simulink model "SistemaP4"  (R2020b)
settings: Solver=ode15s  StartTime=0  StopTime=10  MaxStep=1E-2  RelTol=1e-3
libraries: fl_lib x14, nesl_utility x6, pid_lib x1
settings Model: Creator=ggjai  LastModifiedBy=ggjai
settings SolverCC: AlgebraicLoopSolver=LineSearch
settings DataIOCC: SaveFormat=Array  SaveOutput=off  SignalLogging=off  DSMLogging=off  ReturnWorkspaceOutputs=off  TimeSaveName=t
settings DebuggingCC: AlgebraicLoopMsg=none  ArtificialAlgebraicLoopMsg=none  MaxConsecutiveZCsMsg=none  ModelReferenceExtraNoncontSigs=none  OperatingPointInterfaceChecksumMismatchMsg=none

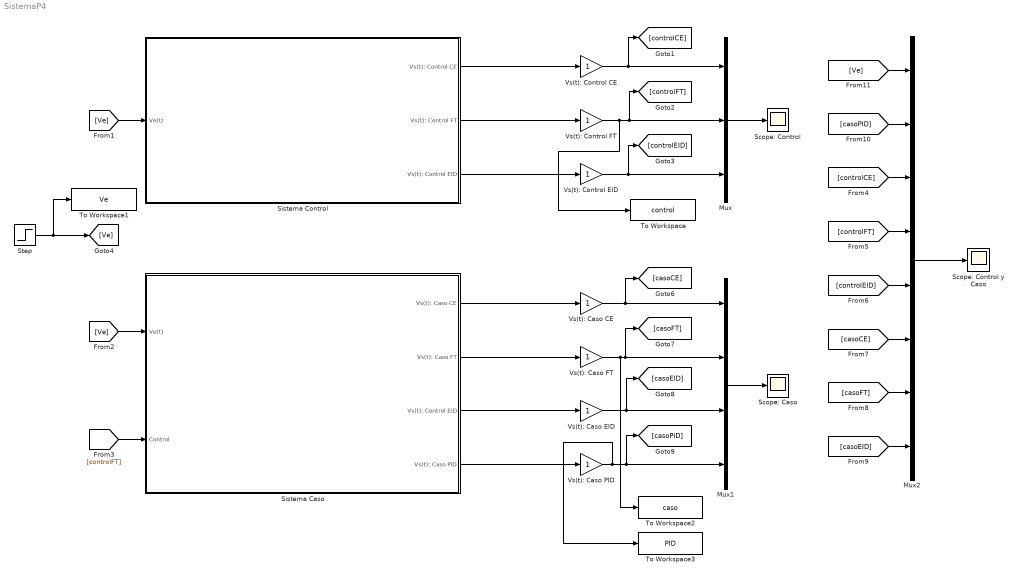
== system SistemaP4 ==
  Mux : Mux  Inputs=3
  Mux1 : Mux
  Mux2 : Mux  Inputs=8
  Scope: Caso : Scope
  Scope: Control : Scope
  Scope: Control y Caso : Scope
  Sistema Caso : Subsystem
  Sistema Control : Subsystem
  Step : Step  SampleTime=0
  To Workspace : ToWorkspace  VariableName=control  SampleTime=-1
  To Workspace1 : ToWorkspace  VariableName=Ve  SampleTime=-1
  To Workspace2 : ToWorkspace  VariableName=caso  SampleTime=-1
  To Workspace3 : ToWorkspace  VariableName=PID  SampleTime=-1
  Vs(t): Caso CE : Gain
  Vs(t): Caso EID : Gain
  Vs(t): Caso FT : Gain
  Vs(t): Caso PID : Gain
  Vs(t): Control CE : Gain
  Vs(t): Control EID : Gain
  Vs(t): Control FT : Gain
  wires:
  [Ve] -> Sistema Control/1(Ve(t))
  Mux/1 -> Scope: Control/1
  Step/1 -> To Workspace1/1, [Ve]
  Sistema Control/3(Vs(t): Control EID) -> Vs(t): Control EID/1
  Vs(t): Control EID/1 -> [controlEID], Mux/3
  Vs(t): Control FT/1 -> To Workspace/1, [controlFT], Mux/2
  Sistema Control/2(Vs(t): Control FT) -> Vs(t): Control FT/1
  Sistema Control/1(Vs(t): Control CE) -> Vs(t): Control CE/1
  Vs(t): Control CE/1 -> [controlCE], Mux/1
  [Ve] -> Sistema Caso/1(Ve(t))
  Mux1/1 -> Scope: Caso/1
  Vs(t): Caso CE/1 -> [casoCE], Mux1/1
  Vs(t): Caso FT/1 -> To Workspace2/1, [casoFT], Mux1/2
  Vs(t): Caso EID/1 -> [casoEID], Mux1/3
  Sistema Caso/1(Vs(t): Caso CE) -> Vs(t): Caso CE/1
  Sistema Caso/2(Vs(t): Caso FT) -> Vs(t): Caso FT/1
  Sistema Caso/3(Vs(t): Control EID) -> Vs(t): Caso EID/1
  Mux2/1 -> Scope: Control y Caso/1
  Sistema Caso/4(Vs(t): Caso PID) -> Vs(t): Caso PID/1
  Vs(t): Caso PID/1 -> To Workspace3/1, Mux1/4, [casoPID]
  [controlFT] -> Sistema Caso/2(Control)
  [casoEID] -> Mux2/8
  [casoFT] -> Mux2/7
  [casoCE] -> Mux2/6
  [controlEID] -> Mux2/5
  [controlFT] -> Mux2/4
  [controlCE] -> Mux2/3
  [casoPID] -> Mux2/2
  [Ve] -> Mux2/1

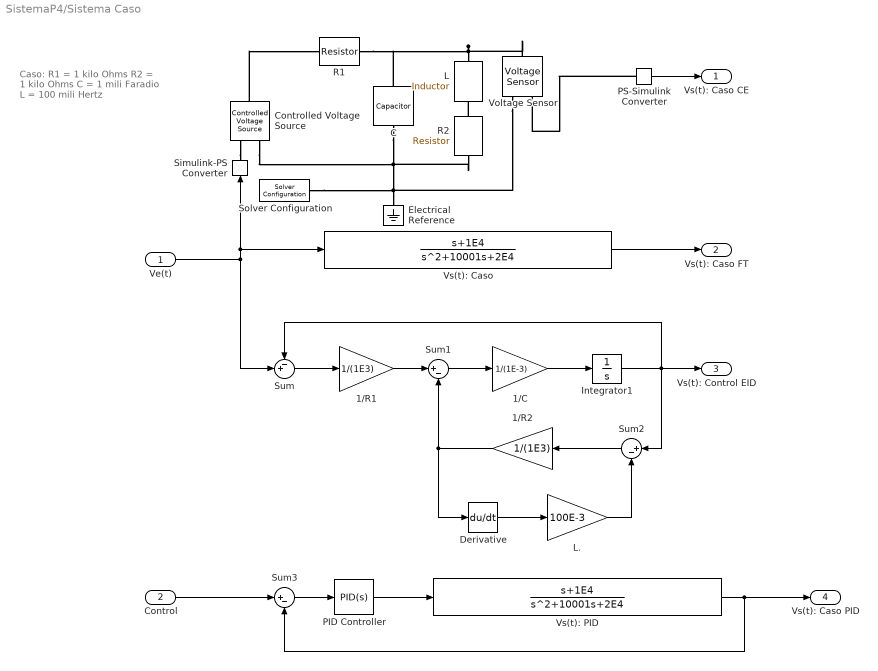
== system SistemaP4/Sistema Caso ==
  note: Caso:
      | R1 = 1 kilo Ohms
      | R2 = 1 kilo Ohms
      | C = 1 mili Faradio
      | L = 100 mili Hertz
  Ve(t) : Inport
  Control : Inport  Port=2
  1/C : Gain  Gain=1/(1E-3)
  1/R1 : Gain  Gain=1/(1E3)
  1/R2 : Gain  Gain=1/(1E3)
  C : fl_lib/Electrical/Electrical Elements/Capacitor  c=1 mF  r=1e-6 Ohm  g=0 1/Ohm  i_specify=off  i_priority=None  i=0 A  i_nominal_specify=off  i_nominal_unit=A  i_nominal_value=1  v_specify=off  v_priority=None  v=0 V  v_nominal_specify=off  v_nominal_unit=V  v_nominal_value=1  vc_specify=off  vc_priority=High  vc=0 V  vc_nominal_specify=off  vc_nominal_unit=V  vc_nominal_value=1
  Controlled Voltage Source : fl_lib/Electrical/Electrical Sources/Controlled Voltage Source
  Derivative : Derivative
  Electrical Reference : fl_lib/Electrical/Electrical Elements/Electrical Reference
  Integrator1 : Integrator
  L : fl_lib/Electrical/Electrical Elements/Inductor  l=100 mH  r=0 Ohm  g=1e-9 1/Ohm  i_specify=off  i_priority=None  i=0 A  i_nominal_specify=off  i_nominal_unit=A  i_nominal_value=1  v_specify=off  v_priority=None  v=0 V  v_nominal_specify=off  v_nominal_unit=V  v_nominal_value=1  i_L_specify=off  i_L_priority=High  i_L=0 A  i_L_nominal_specify=off  i_L_nominal_unit=A  i_L_nominal_value=1
  L. : Gain  Gain=100E-3
  PID Controller : pid_lib/PID Controller  Controller=PID  Form=Parallel  TimeDomain=Continuous-time  UseExternalTs=off  SampleTime=-1  IntegratorMethod=Forward Euler  FilterMethod=Forward Euler  ControllerParametersSource=internal  P=1672.0326  I=517743.8105  D=0.18001  UseFilter=on  N=6391.6622  TunerSelectOption=Transfer Function Based (PID Tuner App)  InitialConditionSource=internal  InitialConditionForIntegrator=0  InitialConditionForFilter=0  DifferentiatorICPrevScaledInput=0  ExternalReset=none  TrackingMode=off  Kt=1  LimitOutput=off  SatLimitsSource=internal  UpperSaturationLimit=inf  LowerSaturationLimit=-inf  LinearizeAsGain=on  AntiWindupMode=none  Kb=1  POutMin=[]  POutMax=[]  IOutMin=[]  IOutMax=[]  DOutMin=[]  DOutMax=[]  NOutMin=[]  NOutMax=[]  SumOutMin=[]  SumOutMax=[]  SaturationOutMin=[]  SaturationOutMax=[]  PParamMin=[]  PParamMax=[]  IParamMin=[]  IParamMax=[]  DParamMin=[]  DParamMax=[]  NParamMin=[]  NParamMax=[]  KbParamMin=[]  KbParamMax=[]  KtParamMin=[]  KtParamMax=[]  KbOutMin=[]  KbOutMax=[]  KtOutMin=[]  KtOutMax=[]  IntegratorOutMin=[]  IntegratorOutMax=[]  FilterOutMin=[]  FilterOutMax=[]  SumI1OutMin=[]  SumI1OutMax=[]  SumI2OutMin=[]  SumI2OutMax=[]  SumI3OutMin=[]  SumI3OutMax=[]  SumI4OutMin=[]  SumI4OutMax=[]  SumDOutMin=[]  SumDOutMax=[]  DifferentiatorOutMin=[]  DifferentiatorOutMax=[]  FilterDiffOutCoefMin=[]  FilterDiffOutCoefMax=[]  ReciprocalOutMin=[]  ReciprocalOutMax=[]  SumDenOutMin=[]  SumDenOutMax=[]  SumNumOutMin=[]  SumNumOutMax=[]  DivideOutMin=[]  DivideOutMax=[]  UdiffTsProdOutMin=[]  UdiffTsProdOutMax=[]  NTsProdOutMin=[]  NTsProdOutMax=[]  UintegralTsProdOutMin=[]  UintegralTsProdOutMax=[]  UngainTsProdOutMin=[]  UngainTsProdOutMax=[]  IntegratorContinuousStateAttributes=''  IntegratorStateMustResolveToSignalObject=off  IntegratorRTWStateStorageClass=Auto  FilterContinuousStateAttributes=''  FilterStateMustResolveToSignalObject=off  FilterRTWStateStorageClass=Auto  ParallelPVariant=InternalParameters  IdealPVariant=Disabled  IVariant=InternalParameters  DVariant=InternalParameters  IntegratorVariant=Continuous  SatVariant=Disabled  AWVariant=Passthrough  PCopyVariant=Disabled  TRVariant=Disabled  FdbkBlocksVariant=Forward  IdealPFdbkVariant=Disabled  SatFdbkVariant=Disabled  DerivativeFilterVariant=ContFilter  NVariant=InternalParameters  NCopyVariant=Disabled  FilterICVariant=InternalICsFilter  IntegratorICVariant=InternalICs  ExternalResetVariant=Disabled  TRSumVariant=Passthrough  SumFdbkVariant=Disabled  SumVariant=Sum_PID  TsampFilterVariant=InternalTs  TsampNgainVariant=Passthrough  TsampIntegralVariant=Passthrough  ExternalSaturationOutDataTypeStr=Inherit: Same as second input
  PS-Simulink Converter : nesl_utility/PS-Simulink Converter  PhysicalDomain=network_engine_domain  SubClassName=ps_output  LeftPortType=input  RightPortType=output  PseudoPeriodic=off  Frequencies=[]  Unit=inherit  AffineConversion=off
  R1 : fl_lib/Electrical/Electrical Elements/Resistor  R=1 kOhm  i_specify=off  i_priority=None  i=0 A  i_nominal_specify=off  i_nominal_unit=A  i_nominal_value=1  v_specify=off  v_priority=None  v=0 V  v_nominal_specify=off  v_nominal_unit=V  v_nominal_value=1
  R2 : fl_lib/Electrical/Electrical Elements/Resistor  R=1 kOhm  i_specify=off  i_priority=None  i=0 A  i_nominal_specify=off  i_nominal_unit=A  i_nominal_value=1  v_specify=off  v_priority=None  v=0 V  v_nominal_specify=off  v_nominal_unit=V  v_nominal_value=1
  Simulink-PS Converter : nesl_utility/Simulink-PS Converter  PhysicalDomain=network_engine_domain  SubClassName=ps_input  LeftPortType=input  RightPortType=output  PseudoPeriodic=off  Frequencies=[]  NoiseDistribution=none  NoiseParameters=[]  Unit=1  AffineConversion=off  FilteringAndDerivatives=provide  SimscapeFilterOrder=1  InputFilterTimeConstant=0.001  UdotUserProvided=0
  Solver Configuration : nesl_utility/Solver Configuration  PhysicalDomain=network_engine_domain  SubClassName=solver  LeftPortType=input  RightPortType=generic  Tones=[]  Harmonics=[]  SimulateNoise=off  Profile=off  UseLocalSampling=off  EnableSwitchedLinearOptims=on  FrequencyDomain=off  UseCCode=off  RelTol=0.001  AbsTol=1e-06  MinStep=1e-09  ToWorkspace=off  RevertToSquareIcSolve=off  NumHomotopyIterations=100  PhasorMode=off  PhasorModeNumHarmonics=1  DoDC=off  ResidualTolerance=1e-09  UseLocalSolver=off  LocalSolverChoice=NE_BACKWARD_EULER_ADVANCER  LocalSolverSampleTime=0.001  DoFixedCost=off  MaxNonlinIter=3  MaxModeIter=2  ComputeImpulses=off  ImpulseIterations=2  LinearAlgebra=auto  EquationFormulation=NE_TIME_EF  DelaysMemoryBudget=1024  AutomaticFiltering=on  FilteringTimeConstant=0.001  PartitionStorageMethod=AS_NEEDED  PartitionMemoryBudget=1024  PartitionMethod=ROBUST
  Sum : Sum  Inputs=-+|
  Sum1 : Sum  Inputs=|+-
  Sum2 : Sum  Inputs=|+-
  Sum3 : Sum  Inputs=|+-
  Voltage Sensor : fl_lib/Electrical/Electrical Sensors/Voltage Sensor
  Vs(t): Caso : TransferFcn  Numerator=[1,1E4]  Denominator=[1,10001,2E4]
  Vs(t): PID : TransferFcn  Numerator=[1,1E4]  Denominator=[1,10001,2E4]
  Vs(t): Caso CE : Outport
  Vs(t): Caso FT : Outport  Port=2
  Vs(t): Control EID : Outport  Port=3
  Vs(t): Caso PID : Outport  Port=4
  wires:
  Ve(t)/1 -> Simulink-PS Converter/1, Vs(t): Caso/1, Sum/2
  PS-Simulink Converter/1 -> Vs(t): Caso CE/1
  Vs(t): Caso/1 -> Vs(t): Caso FT/1
  1/C/1 -> Integrator1/1
  Sum/1 -> 1/R1/1
  Integrator1/1 -> Sum2/1, Vs(t): Control EID/1, Sum/1
  1/R1/1 -> Sum1/1
  Sum1/1 -> 1/C/1
  1/R2/1 -> Derivative/1, Sum1/2
  Sum2/1 -> 1/R2/1
  L./1 -> Sum2/2
  Derivative/1 -> L./1
  Sum3/1 -> PID Controller/1
  PID Controller/1 -> Vs(t): PID/1
  Vs(t): PID/1 -> Vs(t): Caso PID/1, Sum3/2
  Control/1 -> Sum3/1
  connections:
  Controlled Voltage Source/RConn1 -- Simulink-PS Converter/RConn1
  PS-Simulink Converter/LConn1 -- Voltage Sensor/RConn1
  Controlled Voltage Source/LConn1 -- R1/LConn1
  R2/RConn1 -- C/RConn1 -- Controlled Voltage Source/RConn2 -- Solver Configuration/RConn1 -- Electrical Reference/LConn1 -- Voltage Sensor/RConn2
  R2/LConn1 -- L/RConn1
  L/LConn1 -- C/LConn1 -- R1/RConn1 -- Voltage Sensor/LConn1

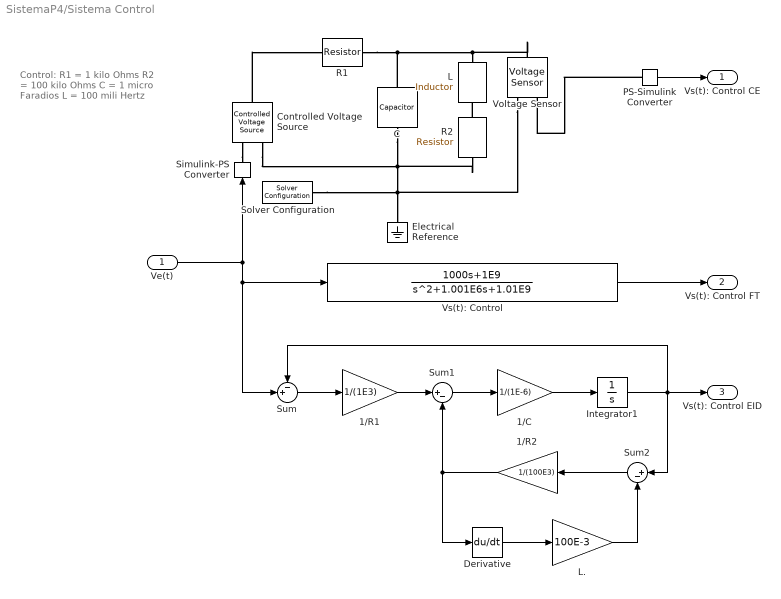
== system SistemaP4/Sistema Control ==
  note: Control:
      | R1 = 1 kilo Ohms
      | R2 = 100 kilo Ohms
      | C = 1 micro Faradios
      | L = 100 mili Hertz
  Ve(t) : Inport
  1/C : Gain  Gain=1/(1E-6)
  1/R1 : Gain  Gain=1/(1E3)
  1/R2 : Gain  Gain=1/(100E3)
  C : fl_lib/Electrical/Electrical Elements/Capacitor  c=1 uF  r=1e-6 Ohm  g=0 1/Ohm  i_specify=off  i_priority=None  i=0 A  i_nominal_specify=off  i_nominal_unit=A  i_nominal_value=1  v_specify=off  v_priority=None  v=0 V  v_nominal_specify=off  v_nominal_unit=V  v_nominal_value=1  vc_specify=off  vc_priority=High  vc=0 V  vc_nominal_specify=off  vc_nominal_unit=V  vc_nominal_value=1
  Controlled Voltage Source : fl_lib/Electrical/Electrical Sources/Controlled Voltage Source
  Derivative : Derivative
  Electrical Reference : fl_lib/Electrical/Electrical Elements/Electrical Reference
  Integrator1 : Integrator
  L : fl_lib/Electrical/Electrical Elements/Inductor  l=100 mH  r=0 Ohm  g=1e-9 1/Ohm  i_specify=off  i_priority=None  i=0 A  i_nominal_specify=off  i_nominal_unit=A  i_nominal_value=1  v_specify=off  v_priority=None  v=0 V  v_nominal_specify=off  v_nominal_unit=V  v_nominal_value=1  i_L_specify=off  i_L_priority=High  i_L=0 A  i_L_nominal_specify=off  i_L_nominal_unit=A  i_L_nominal_value=1
  L. : Gain  Gain=100E-3
  PS-Simulink Converter : nesl_utility/PS-Simulink Converter  PhysicalDomain=network_engine_domain  SubClassName=ps_output  LeftPortType=input  RightPortType=output  PseudoPeriodic=off  Frequencies=[]  Unit=inherit  AffineConversion=off
  R1 : fl_lib/Electrical/Electrical Elements/Resistor  R=1 kOhm  i_specify=off  i_priority=None  i=0 A  i_nominal_specify=off  i_nominal_unit=A  i_nominal_value=1  v_specify=off  v_priority=None  v=0 V  v_nominal_specify=off  v_nominal_unit=V  v_nominal_value=1
  R2 : fl_lib/Electrical/Electrical Elements/Resistor  R=100 kOhm  i_specify=off  i_priority=None  i=0 A  i_nominal_specify=off  i_nominal_unit=A  i_nominal_value=1  v_specify=off  v_priority=None  v=0 V  v_nominal_specify=off  v_nominal_unit=V  v_nominal_value=1
  Simulink-PS Converter : nesl_utility/Simulink-PS Converter  PhysicalDomain=network_engine_domain  SubClassName=ps_input  LeftPortType=input  RightPortType=output  PseudoPeriodic=off  Frequencies=[]  NoiseDistribution=none  NoiseParameters=[]  Unit=1  AffineConversion=off  FilteringAndDerivatives=provide  SimscapeFilterOrder=1  InputFilterTimeConstant=0.001  UdotUserProvided=0
  Solver Configuration : nesl_utility/Solver Configuration  PhysicalDomain=network_engine_domain  SubClassName=solver  LeftPortType=input  RightPortType=generic  Tones=[]  Harmonics=[]  SimulateNoise=off  Profile=off  UseLocalSampling=off  EnableSwitchedLinearOptims=on  FrequencyDomain=off  UseCCode=off  RelTol=0.001  AbsTol=1e-06  MinStep=1e-09  ToWorkspace=off  RevertToSquareIcSolve=off  NumHomotopyIterations=100  PhasorMode=off  PhasorModeNumHarmonics=1  DoDC=off  ResidualTolerance=1e-09  UseLocalSolver=off  LocalSolverChoice=NE_BACKWARD_EULER_ADVANCER  LocalSolverSampleTime=0.001  DoFixedCost=off  MaxNonlinIter=3  MaxModeIter=2  ComputeImpulses=off  ImpulseIterations=2  LinearAlgebra=auto  EquationFormulation=NE_TIME_EF  DelaysMemoryBudget=1024  AutomaticFiltering=on  FilteringTimeConstant=0.001  PartitionStorageMethod=AS_NEEDED  PartitionMemoryBudget=1024  PartitionMethod=ROBUST
  Sum : Sum  Inputs=-+|
  Sum1 : Sum  Inputs=|+-
  Sum2 : Sum  Inputs=|+-
  Voltage Sensor : fl_lib/Electrical/Electrical Sensors/Voltage Sensor
  Vs(t): Control : TransferFcn  Numerator=[1000,1E9]  Denominator=[1,1.001E6,1.01E9]
  Vs(t): Control CE : Outport
  Vs(t): Control FT : Outport  Port=2
  Vs(t): Control EID : Outport  Port=3
  wires:
  Ve(t)/1 -> Sum/2, Vs(t): Control/1, Simulink-PS Converter/1
  PS-Simulink Converter/1 -> Vs(t): Control CE/1
  Vs(t): Control/1 -> Vs(t): Control FT/1
  1/R1/1 -> Sum1/1
  Sum1/1 -> 1/C/1
  1/C/1 -> Integrator1/1
  Integrator1/1 -> Sum2/1, Vs(t): Control EID/1, Sum/1
  Sum/1 -> 1/R1/1
  1/R2/1 -> Derivative/1, Sum1/2
  Derivative/1 -> L./1
  L./1 -> Sum2/2
  Sum2/1 -> 1/R2/1
  connections:
  Controlled Voltage Source/RConn1 -- Simulink-PS Converter/RConn1
  PS-Simulink Converter/LConn1 -- Voltage Sensor/RConn1
  Controlled Voltage Source/LConn1 -- R1/LConn1
  Controlled Voltage Source/RConn2 -- R2/RConn1 -- Voltage Sensor/RConn2 -- Solver Configuration/RConn1 -- Electrical Reference/LConn1 -- C/RConn1
  R2/LConn1 -- L/RConn1
  R1/RConn1 -- C/LConn1 -- Voltage Sensor/LConn1 -- L/LConn1
